simulink model "foc_current_loops"  (R2026b)
settings: Solver=VariableStepAuto  StopTime=6
values from neighbouring files (symbols this model uses):
  D = 5e-5    (= 5e-05)    [setup_foc_current.m]
  J = 0.0239    [setup_foc_current.m]
  Ki_i = 150.0    (= 150)    [setup_foc_current.m]
  Ki_w = 10.0    (= 10)    [setup_foc_current.m]
  Kp_i = 1.5    [setup_foc_current.m]
  Kp_w = 2.0    (= 2)    [setup_foc_current.m]
  L = (Ld + Lq) / 2    (= 0.000225)    [setup_foc_current.m]
  P = 10    [setup_foc_current.m]
  phi_m = 0.05867    [setup_foc_current.m]
  Rs = 25.68e-3    (= 0.02568)    [setup_foc_current.m]
  V_pico = 48    [setup_foc_current.m]
libraries: slpidlib x3, simulink x2
settings Model: Creator=Lemão Som  LastModifiedBy=Lemão Som

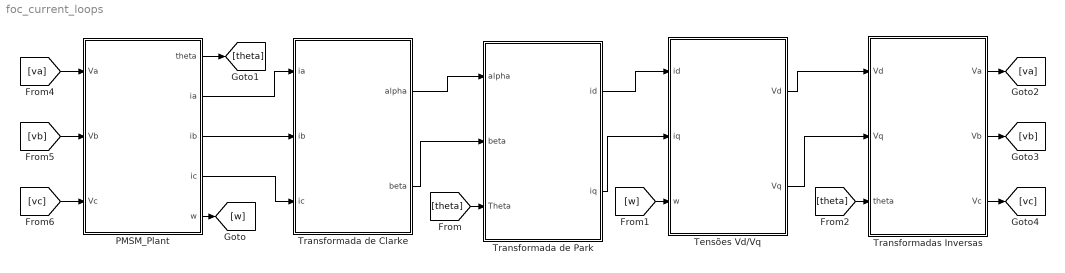
== system foc_current_loops ==
  PMSM_Plant : Subsystem
  Tensões Vd/Vq : Subsystem
  Transformada de Clarke : Subsystem
  Transformada de Park : Subsystem
  Transformadas Inversas : Subsystem
  wires:
  [va] -> PMSM_Plant/1(Va)
  [vb] -> PMSM_Plant/2(Vb)
  [vc] -> PMSM_Plant/3(Vc)
  PMSM_Plant/2(ia) -> Transformada de Clarke/1(ia)
  PMSM_Plant/3(ib) -> Transformada de Clarke/2(ib)
  PMSM_Plant/4(ic) -> Transformada de Clarke/3(ic)
  Transformada de Clarke/1(alpha) -> Transformada de Park/1(alpha)
  PMSM_Plant/5(w) -> [w]
  PMSM_Plant/1(theta) -> [theta]
  [theta] -> Transformada de Park/3(Theta)
  [w] -> Tensões Vd/Vq/3(w)
  Tensões Vd/Vq/1(Vd) -> Transformadas Inversas/1(Vd)
  Tensões Vd/Vq/2(Vq) -> Transformadas Inversas/2(Vq)
  [theta] -> Transformadas Inversas/3(theta)
  Transformadas Inversas/1(Va) -> [va]
  Transformadas Inversas/2(Vb) -> [vb]
  Transformadas Inversas/3(Vc) -> [vc]
  Transformada de Clarke/2(beta) -> Transformada de Park/2(beta)
  Transformada de Park/2(iq) -> Tensões Vd/Vq/2(iq)
  Transformada de Park/1(id) -> Tensões Vd/Vq/1(id)

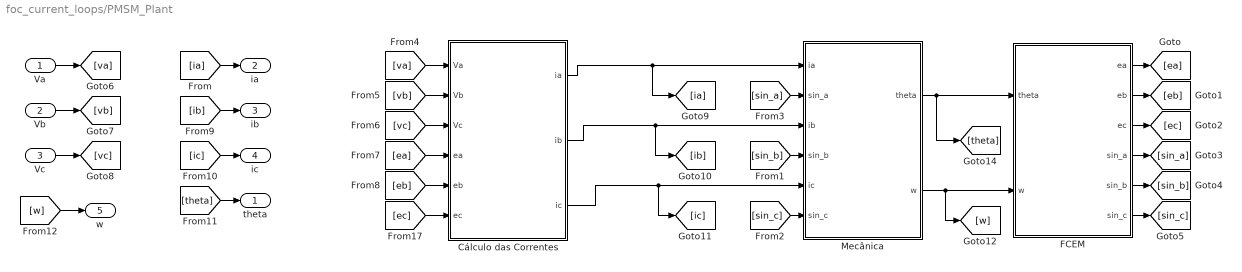
== system foc_current_loops/PMSM_Plant ==
  Va : Inport
  Vb : Inport  Port=2
  Vc : Inport  Port=3
  Cálculo das Correntes : Subsystem
  FCEM : Subsystem
  Mecânica : Subsystem
  theta : Outport
  ia : Outport  Port=2
  ib : Outport  Port=3
  ic : Outport  Port=4
  w : Outport  Port=5
  wires:
  FCEM/2(eb) -> [eb]
  [sin_a] -> Mecânica/2(sin_a)
  [ea] -> Cálculo das Correntes/4(ea)
  [va] -> Cálculo das Correntes/1(Va)
  Cálculo das Correntes/3(ic) -> [ic], Mecânica/5(ic)
  [vb] -> Cálculo das Correntes/2(Vb)
  FCEM/4(sin_a) -> [sin_a]
  FCEM/1(ea) -> [ea]
  Mecânica/1(theta) -> [theta], FCEM/1(theta)
  [vc] -> Cálculo das Correntes/3(Vc)
  FCEM/5(sin_b) -> [sin_b]
  Cálculo das Correntes/2(ib) -> [ib], Mecânica/3(ib)
  Mecânica/2(w) -> [w], FCEM/2(w)
  Cálculo das Correntes/1(ia) -> [ia], Mecânica/1(ia)
  [sin_b] -> Mecânica/4(sin_b)
  [ec] -> Cálculo das Correntes/6(ec)
  [eb] -> Cálculo das Correntes/5(eb)
  FCEM/6(sin_c) -> [sin_c]
  FCEM/3(ec) -> [ec]
  [sin_c] -> Mecânica/6(sin_c)
  Va/1 -> [va]
  Vb/1 -> [vb]
  Vc/1 -> [vc]
  [ia] -> ia/1
  [ib] -> ib/1
  [ic] -> ic/1
  [w] -> w/1
  [theta] -> theta/1

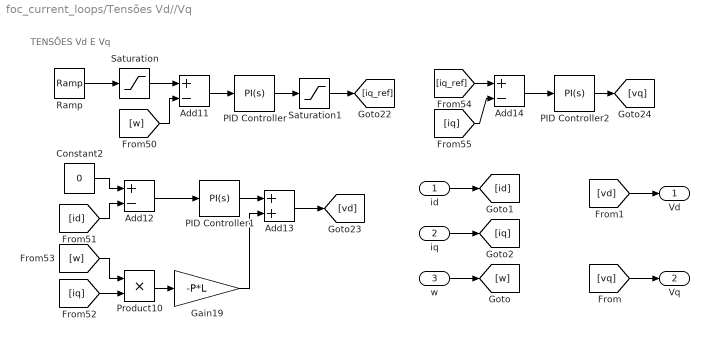
== system foc_current_loops/Tensões Vd//Vq ==
  note: TENSÕES Vd E Vq
  id : Inport
  iq : Inport  Port=2
  w : Inport  Port=3
  Add11 : Sum  Inputs=+-
  Add12 : Sum  Inputs=+-
  Add13 : Sum
  Add14 : Sum  Inputs=+-
  Constant2 : Constant  Value=0
  Gain19 : Gain  Gain=-P*L
  PID Controller : slpidlib/PID Controller  Controller=PI  Form=Parallel  TimeDomain=Continuous-time  UseExternalTs=off  SampleTime=-1  IntegratorMethod=Forward Euler  FilterMethod=Forward Euler  ControllerParametersSource=internal  P=Kp_w  I=Ki_w  UseKiTs=off  D=0  UseExternalDerivativeSource=off  N=100  UseFilter=on  TunerSelectOption=Transfer Function Based (PID Tuner App)  InitialConditionSource=internal  InitialConditionForIntegrator=0  InitialConditionForFilter=0  DifferentiatorICPrevScaledInput=0  ExternalReset=none  TrackingMode=off  Kt=1  LimitOutput=off  SatLimitsSource=internal  UpperSaturationLimit=inf  LowerSaturationLimit=-inf  LinearizeAsGain=on  AntiWindupMode=none  Kb=1  LimitIntegrator=off  UpperIntegratorSaturationLimit=inf  LowerIntegratorSaturationLimit=-inf  POutMin=[]  POutMax=[]  IOutMin=[]  IOutMax=[]  DOutMin=[]  DOutMax=[]  NOutMin=[]  NOutMax=[]  SumOutMin=[]  SumOutMax=[]  SaturationOutMin=[]  SaturationOutMax=[]  PParamMin=[]  PParamMax=[]  IParamMin=[]  IParamMax=[]  DParamMin=[]  DParamMax=[]  NParamMin=[]  NParamMax=[]  KbParamMin=[]  KbParamMax=[]  KtParamMin=[]  KtParamMax=[]  KbOutMin=[]  KbOutMax=[]  KtOutMin=[]  KtOutMax=[]  IntegratorOutMin=[]  IntegratorOutMax=[]  FilterOutMin=[]  FilterOutMax=[]  SumI1OutMin=[]  SumI1OutMax=[]  SumI2OutMin=[]  SumI2OutMax=[]  SumI3OutMin=[]  SumI3OutMax=[]  SumI4OutMin=[]  SumI4OutMax=[]  SumDOutMin=[]  SumDOutMax=[]  DifferentiatorOutMin=[]  DifferentiatorOutMax=[]  FilterDiffOutCoefMin=[]  FilterDiffOutCoefMax=[]  ReciprocalOutMin=[]  ReciprocalOutMax=[]  SumDenOutMin=[]  SumDenOutMax=[]  SumNumOutMin=[]  SumNumOutMax=[]  DivideOutMin=[]  DivideOutMax=[]  UdiffTsProdOutMin=[]  UdiffTsProdOutMax=[]  NTsProdOutMin=[]  NTsProdOutMax=[]  UintegralTsProdOutMin=[]  UintegralTsProdOutMax=[]  UngainTsProdOutMin=[]  UngainTsProdOutMax=[]  ClampingZeroOutDataTypeStr=Inherit: Inherit via back propagation  ClampingZeroOutMin=[]  ClampingZeroOutMax=[]  FilterDenConstantOutDataTypeStr=Inherit: Inherit via back propagation  FilterDenConstantOutMin=[]  FilterDenConstantOutMax=[]  PCopyOutDataTypeStr=Inherit: Inherit via back propagation  PCopyOutMin=[]  PCopyOutMax=[]  NCopyOutDataTypeStr=Inherit: Inherit via back propagation  NCopyOutMin=[]  NCopyOutMax=[]  IntegratorContinuousStateAttributes=''  IntegratorStateMustResolveToSignalObject=off  IntegratorRTWStateStorageClass=Auto  FilterContinuousStateAttributes=''  FilterStateMustResolveToSignalObject=off  FilterRTWStateStorageClass=Auto  ParallelPVariant=InternalParameters  IdealPVariant=Disabled  IVariant=InternalParameters  DVariant=Disabled  IntegratorVariant=Continuous  SatVariant=Disabled  AWVariant=Passthrough  PCopyVariant=Disabled  TRVariant=Disabled  FdbkBlocksVariant=Forward  IdealPFdbkVariant=Disabled  SatFdbkVariant=Disabled  DerivativeFilterVariant=Disabled  NVariant=Disabled  NCopyVariant=Disabled_SignalSpec  FilterICVariant=Disabled  IntegratorICVariant=InternalICs  ExternalResetVariant=Disabled  TRSumVariant=Passthrough  SumFdbkVariant=Disabled  SumVariant=Sum_PI  TsampFilterVariant=InternalTs  TsampNgainVariant=Passthrough  TsampIntegralVariant=Disabled_SignalSpec  ExternalSaturationOutDataTypeStr=Inherit: Same as second input  DerivativeSourceVariant=Disabled  PreIntVariant=InternalPreInt
  PID Controller1 : slpidlib/PID Controller  Controller=PI  Form=Parallel  TimeDomain=Continuous-time  UseExternalTs=off  SampleTime=-1  IntegratorMethod=Forward Euler  FilterMethod=Forward Euler  ControllerParametersSource=internal  P=Kp_i  I=Ki_i  UseKiTs=off  D=0  UseExternalDerivativeSource=off  N=100  UseFilter=on  TunerSelectOption=Transfer Function Based (PID Tuner App)  InitialConditionSource=internal  InitialConditionForIntegrator=0  InitialConditionForFilter=0  DifferentiatorICPrevScaledInput=0  ExternalReset=none  TrackingMode=off  Kt=1  LimitOutput=off  SatLimitsSource=internal  UpperSaturationLimit=inf  LowerSaturationLimit=-inf  LinearizeAsGain=on  AntiWindupMode=none  Kb=1  LimitIntegrator=off  UpperIntegratorSaturationLimit=inf  LowerIntegratorSaturationLimit=-inf  POutMin=[]  POutMax=[]  IOutMin=[]  IOutMax=[]  DOutMin=[]  DOutMax=[]  NOutMin=[]  NOutMax=[]  SumOutMin=[]  SumOutMax=[]  SaturationOutMin=[]  SaturationOutMax=[]  PParamMin=[]  PParamMax=[]  IParamMin=[]  IParamMax=[]  DParamMin=[]  DParamMax=[]  NParamMin=[]  NParamMax=[]  KbParamMin=[]  KbParamMax=[]  KtParamMin=[]  KtParamMax=[]  KbOutMin=[]  KbOutMax=[]  KtOutMin=[]  KtOutMax=[]  IntegratorOutMin=[]  IntegratorOutMax=[]  FilterOutMin=[]  FilterOutMax=[]  SumI1OutMin=[]  SumI1OutMax=[]  SumI2OutMin=[]  SumI2OutMax=[]  SumI3OutMin=[]  SumI3OutMax=[]  SumI4OutMin=[]  SumI4OutMax=[]  SumDOutMin=[]  SumDOutMax=[]  DifferentiatorOutMin=[]  DifferentiatorOutMax=[]  FilterDiffOutCoefMin=[]  FilterDiffOutCoefMax=[]  ReciprocalOutMin=[]  ReciprocalOutMax=[]  SumDenOutMin=[]  SumDenOutMax=[]  SumNumOutMin=[]  SumNumOutMax=[]  DivideOutMin=[]  DivideOutMax=[]  UdiffTsProdOutMin=[]  UdiffTsProdOutMax=[]  NTsProdOutMin=[]  NTsProdOutMax=[]  UintegralTsProdOutMin=[]  UintegralTsProdOutMax=[]  UngainTsProdOutMin=[]  UngainTsProdOutMax=[]  ClampingZeroOutDataTypeStr=Inherit: Inherit via back propagation  ClampingZeroOutMin=[]  ClampingZeroOutMax=[]  FilterDenConstantOutDataTypeStr=Inherit: Inherit via back propagation  FilterDenConstantOutMin=[]  FilterDenConstantOutMax=[]  PCopyOutDataTypeStr=Inherit: Inherit via back propagation  PCopyOutMin=[]  PCopyOutMax=[]  NCopyOutDataTypeStr=Inherit: Inherit via back propagation  NCopyOutMin=[]  NCopyOutMax=[]  IntegratorContinuousStateAttributes=''  IntegratorStateMustResolveToSignalObject=off  IntegratorRTWStateStorageClass=Auto  FilterContinuousStateAttributes=''  FilterStateMustResolveToSignalObject=off  FilterRTWStateStorageClass=Auto  ParallelPVariant=InternalParameters  IdealPVariant=Disabled  IVariant=InternalParameters  DVariant=Disabled  IntegratorVariant=Continuous  SatVariant=Disabled  AWVariant=Passthrough  PCopyVariant=Disabled  TRVariant=Disabled  FdbkBlocksVariant=Forward  IdealPFdbkVariant=Disabled  SatFdbkVariant=Disabled  DerivativeFilterVariant=Disabled  NVariant=Disabled  NCopyVariant=Disabled_SignalSpec  FilterICVariant=Disabled  IntegratorICVariant=InternalICs  ExternalResetVariant=Disabled  TRSumVariant=Passthrough  SumFdbkVariant=Disabled  SumVariant=Sum_PI  TsampFilterVariant=InternalTs  TsampNgainVariant=Passthrough  TsampIntegralVariant=Disabled_SignalSpec  ExternalSaturationOutDataTypeStr=Inherit: Same as second input  DerivativeSourceVariant=Disabled  PreIntVariant=InternalPreInt
  PID Controller2 : slpidlib/PID Controller  Controller=PI  Form=Parallel  TimeDomain=Continuous-time  UseExternalTs=off  SampleTime=-1  IntegratorMethod=Forward Euler  FilterMethod=Forward Euler  ControllerParametersSource=internal  P=Kp_i  I=Ki_i  UseKiTs=off  D=0  UseExternalDerivativeSource=off  N=100  UseFilter=on  TunerSelectOption=Transfer Function Based (PID Tuner App)  InitialConditionSource=internal  InitialConditionForIntegrator=0  InitialConditionForFilter=0  DifferentiatorICPrevScaledInput=0  ExternalReset=none  TrackingMode=off  Kt=1  LimitOutput=off  SatLimitsSource=internal  UpperSaturationLimit=inf  LowerSaturationLimit=-inf  LinearizeAsGain=on  AntiWindupMode=none  Kb=1  LimitIntegrator=off  UpperIntegratorSaturationLimit=inf  LowerIntegratorSaturationLimit=-inf  POutMin=[]  POutMax=[]  IOutMin=[]  IOutMax=[]  DOutMin=[]  DOutMax=[]  NOutMin=[]  NOutMax=[]  SumOutMin=[]  SumOutMax=[]  SaturationOutMin=[]  SaturationOutMax=[]  PParamMin=[]  PParamMax=[]  IParamMin=[]  IParamMax=[]  DParamMin=[]  DParamMax=[]  NParamMin=[]  NParamMax=[]  KbParamMin=[]  KbParamMax=[]  KtParamMin=[]  KtParamMax=[]  KbOutMin=[]  KbOutMax=[]  KtOutMin=[]  KtOutMax=[]  IntegratorOutMin=[]  IntegratorOutMax=[]  FilterOutMin=[]  FilterOutMax=[]  SumI1OutMin=[]  SumI1OutMax=[]  SumI2OutMin=[]  SumI2OutMax=[]  SumI3OutMin=[]  SumI3OutMax=[]  SumI4OutMin=[]  SumI4OutMax=[]  SumDOutMin=[]  SumDOutMax=[]  DifferentiatorOutMin=[]  DifferentiatorOutMax=[]  FilterDiffOutCoefMin=[]  FilterDiffOutCoefMax=[]  ReciprocalOutMin=[]  ReciprocalOutMax=[]  SumDenOutMin=[]  SumDenOutMax=[]  SumNumOutMin=[]  SumNumOutMax=[]  DivideOutMin=[]  DivideOutMax=[]  UdiffTsProdOutMin=[]  UdiffTsProdOutMax=[]  NTsProdOutMin=[]  NTsProdOutMax=[]  UintegralTsProdOutMin=[]  UintegralTsProdOutMax=[]  UngainTsProdOutMin=[]  UngainTsProdOutMax=[]  ClampingZeroOutDataTypeStr=Inherit: Inherit via back propagation  ClampingZeroOutMin=[]  ClampingZeroOutMax=[]  FilterDenConstantOutDataTypeStr=Inherit: Inherit via back propagation  FilterDenConstantOutMin=[]  FilterDenConstantOutMax=[]  PCopyOutDataTypeStr=Inherit: Inherit via back propagation  PCopyOutMin=[]  PCopyOutMax=[]  NCopyOutDataTypeStr=Inherit: Inherit via back propagation  NCopyOutMin=[]  NCopyOutMax=[]  IntegratorContinuousStateAttributes=''  IntegratorStateMustResolveToSignalObject=off  IntegratorRTWStateStorageClass=Auto  FilterContinuousStateAttributes=''  FilterStateMustResolveToSignalObject=off  FilterRTWStateStorageClass=Auto  ParallelPVariant=InternalParameters  IdealPVariant=Disabled  IVariant=InternalParameters  DVariant=Disabled  IntegratorVariant=Continuous  SatVariant=Disabled  AWVariant=Passthrough  PCopyVariant=Disabled  TRVariant=Disabled  FdbkBlocksVariant=Forward  IdealPFdbkVariant=Disabled  SatFdbkVariant=Disabled  DerivativeFilterVariant=Disabled  NVariant=Disabled  NCopyVariant=Disabled_SignalSpec  FilterICVariant=Disabled  IntegratorICVariant=InternalICs  ExternalResetVariant=Disabled  TRSumVariant=Passthrough  SumFdbkVariant=Disabled  SumVariant=Sum_PI  TsampFilterVariant=InternalTs  TsampNgainVariant=Passthrough  TsampIntegralVariant=Disabled_SignalSpec  ExternalSaturationOutDataTypeStr=Inherit: Same as second input  DerivativeSourceVariant=Disabled  PreIntVariant=InternalPreInt
  Product10 : Product
  Ramp : simulink/Sources/Ramp  slope=600  start=0  InitialOutput=0
  Saturation : Saturate  UpperLimit=300  LowerLimit=0
  Saturation1 : Saturate  UpperLimit=250  LowerLimit=-250
  Vd : Outport
  Vq : Outport  Port=2
  wires:
  Add11/1 -> PID Controller/1
  PID Controller2/1 -> [vq]
  Saturation/1 -> Add11/1
  [id] -> Add12/2
  [w] -> Product10/1
  Product10/1 -> Gain19/1
  PID Controller/1 -> Saturation1/1
  [iq] -> Add14/2
  [iq] -> Product10/2
  Add13/1 -> [vd]
  [iq_ref] -> Add14/1
  Add14/1 -> PID Controller2/1
  [w] -> Add11/2
  Gain19/1 -> Add13/2
  PID Controller1/1 -> Add13/1
  Ramp/1 -> Saturation/1
  Add12/1 -> PID Controller1/1
  Constant2/1 -> Add12/1
  Saturation1/1 -> [iq_ref]
  w/1 -> [w]
  id/1 -> [id]
  iq/1 -> [iq]
  [vq] -> Vq/1
  [vd] -> Vd/1

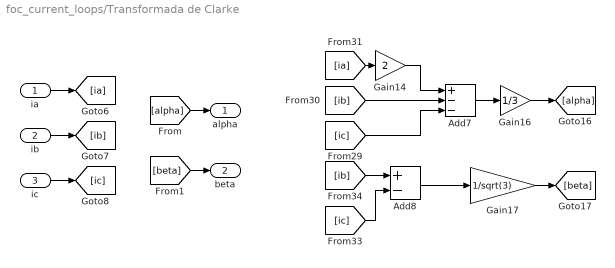
== system foc_current_loops/Transformada de Clarke ==
  ia : Inport
  ib : Inport  Port=2
  ic : Inport  Port=3
  Add7 : Sum  Inputs=+--
  Add8 : Sum  Inputs=+-
  Gain14 : Gain  Gain=2
  Gain16 : Gain  Gain=1/3
  Gain17 : Gain  Gain=1/sqrt(3)
  alpha : Outport
  beta : Outport  Port=2
  wires:
  ic/1 -> [ic]
  ib/1 -> [ib]
  ia/1 -> [ia]
  Gain14/1 -> Add7/1
  [ib] -> Add8/1
  Gain16/1 -> [alpha]
  [ic] -> Add7/3
  Gain17/1 -> [beta]
  [ic] -> Add8/2
  [ia] -> Gain14/1
  Add8/1 -> Gain17/1
  Add7/1 -> Gain16/1
  [ib] -> Add7/2
  [alpha] -> alpha/1
  [beta] -> beta/1

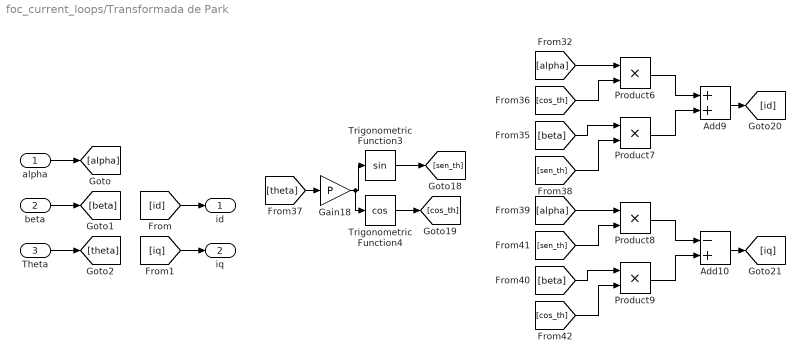
== system foc_current_loops/Transformada de Park ==
  alpha : Inport
  beta : Inport  Port=2
  Theta : Inport  Port=3
  Add10 : Sum  Inputs=-+
  Add9 : Sum
  Gain18 : Gain  Gain=P
  Product{6..9} (4 alike) : Product
  Trigonometric Function3 : Trigonometry
  Trigonometric Function4 : Trigonometry  Operator=cos
  id : Outport
  iq : Outport  Port=2
  wires:
  [iq] -> iq/1
  Theta/1 -> [theta]
  Add10/1 -> [iq]
  Add9/1 -> [id]
  Product7/1 -> Add9/2
  Product6/1 -> Add9/1
  [sen_th] -> Product8/2
  [sen_th] -> Product7/2
  [alpha] -> Product6/1
  [beta] -> Product9/1
  [theta] -> Gain18/1
  Product9/1 -> Add10/2
  Gain18/1 -> Trigonometric Function4/1, Trigonometric Function3/1
  [cos_th] -> Product9/2
  [beta] -> Product7/1
  Trigonometric Function4/1 -> [cos_th]
  alpha/1 -> [alpha]
  [alpha] -> Product8/1
  beta/1 -> [beta]
  [id] -> id/1
  Product8/1 -> Add10/1
  [cos_th] -> Product6/2
  Trigonometric Function3/1 -> [sen_th]

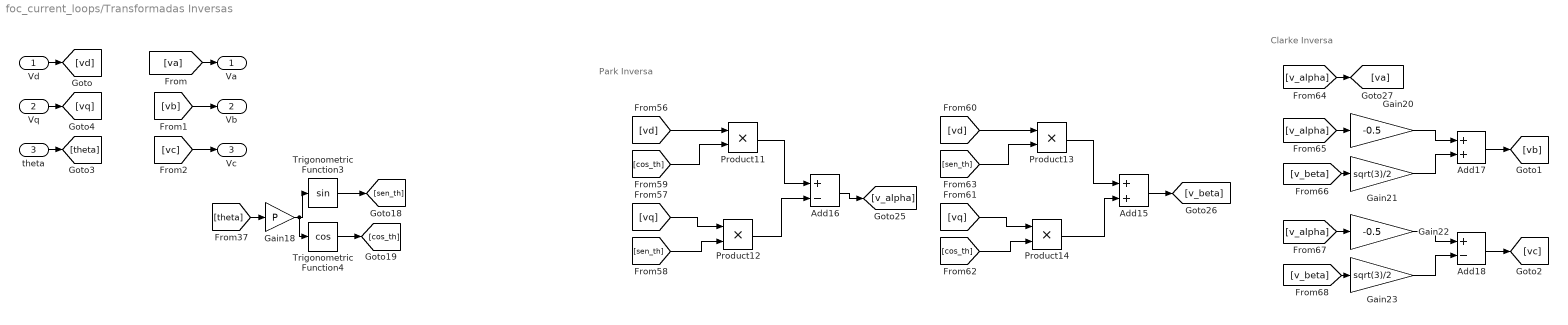
== system foc_current_loops/Transformadas Inversas ==
  note: Clarke Inversa
  note: Park Inversa
  Vd : Inport
  Vq : Inport  Port=2
  theta : Inport  Port=3
  Add15 : Sum
  Add16 : Sum  Inputs=+-
  Add17 : Sum
  Add18 : Sum  Inputs=+-
  Gain18 : Gain  Gain=P
  Gain20 : Gain  Gain=-0.5
  Gain21 : Gain  Gain=sqrt(3)/2
  Gain22 : Gain  Gain=-0.5
  Gain23 : Gain  Gain=sqrt(3)/2
  Product{11..14} (4 alike) : Product
  Trigonometric Function3 : Trigonometry
  Trigonometric Function4 : Trigonometry  Operator=cos
  Va : Outport
  Vb : Outport  Port=2
  Vc : Outport  Port=3
  wires:
  Add15/1 -> [v_beta]
  [cos_th] -> Product11/2
  Gain21/1 -> Add17/2
  [v_alpha] -> Gain22/1
  Add16/1 -> [v_alpha]
  [sen_th] -> Product13/2
  Product11/1 -> Add16/1
  Add18/1 -> [vc]
  [vd] -> Product11/1
  [vd] -> Product13/1
  [v_alpha] -> Gain20/1
  Gain23/1 -> Add18/2
  Gain20/1 -> Add17/1
  Gain22/1 -> Add18/1
  Product12/1 -> Add16/2
  Product14/1 -> Add15/2
  [v_beta] -> Gain21/1
  [vq] -> Product12/1
  [vq] -> Product14/1
  [sen_th] -> Product12/2
  [v_beta] -> Gain23/1
  [v_alpha] -> [va]
  Product13/1 -> Add15/1
  [cos_th] -> Product14/2
  Add17/1 -> [vb]
  Trigonometric Function3/1 -> [sen_th]
  Gain18/1 -> Trigonometric Function4/1, Trigonometric Function3/1
  [theta] -> Gain18/1
  Trigonometric Function4/1 -> [cos_th]
  Vd/1 -> [vd]
  theta/1 -> [theta]
  Vq/1 -> [vq]
  [va] -> Va/1
  [vb] -> Vb/1
  [vc] -> Vc/1

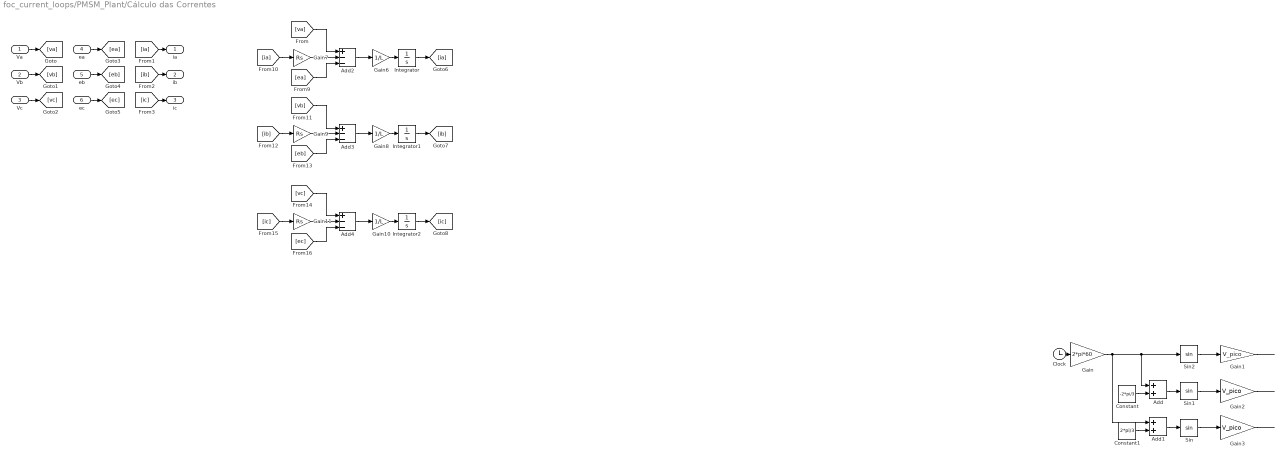
== system foc_current_loops/PMSM_Plant/Cálculo das Correntes ==
  Va : Inport
  Vb : Inport  Port=2
  Vc : Inport  Port=3
  ea : Inport  Port=4
  eb : Inport  Port=5
  ec : Inport  Port=6
  Add : Sum
  Add1 : Sum
  Add2 : Sum  Inputs=+--
  Add3 : Sum  Inputs=+--
  Add4 : Sum  Inputs=+--
  Clock : Clock
  Constant : Constant  Value=-2*pi/3
  Constant1 : Constant  Value=2*pi/3
  Gain : Gain  Gain=2*pi*60
  Gain1 : Gain  Gain=V_pico
  Gain10 : Gain  Gain=1/L
  Gain11 : Gain  Gain=Rs
  Gain2 : Gain  Gain=V_pico
  Gain3 : Gain  Gain=V_pico
  Gain6 : Gain  Gain=1/L
  Gain7 : Gain  Gain=Rs
  Gain8 : Gain  Gain=1/L
  Gain9 : Gain  Gain=Rs
  Integrator : Integrator
  Integrator1 : Integrator
  Integrator2 : Integrator
  Sin : Trigonometry
  Sin1 : Trigonometry
  Sin2 : Trigonometry
  ia : Outport
  ib : Outport  Port=2
  ic : Outport  Port=3
  wires:
  Sin/1 -> Gain3/1
  Clock/1 -> Gain/1
  Gain1/1 -> ?
  Sin1/1 -> Gain2/1
  Gain2/1 -> ?
  Add1/1 -> Sin/1
  Sin2/1 -> Gain1/1
  Gain/1 -> Add/1, Sin2/1, Add1/1
  Gain3/1 -> ?
  Add/1 -> Sin1/1
  Constant/1 -> Add/2
  Constant1/1 -> Add1/2
  Integrator2/1 -> [ic]
  [ea] -> Add2/3
  [ec] -> Add4/3
  Add3/1 -> Gain8/1
  [eb] -> Add3/3
  Integrator1/1 -> [ib]
  Gain7/1 -> Add2/2
  Gain8/1 -> Integrator1/1
  Add4/1 -> Gain10/1
  Add2/1 -> Gain6/1
  Gain10/1 -> Integrator2/1
  [va] -> Add2/1
  [ic] -> Gain11/1
  Gain9/1 -> Add3/2
  [ia] -> Gain7/1
  Integrator/1 -> [ia]
  Gain11/1 -> Add4/2
  [vc] -> Add4/1
  [vb] -> Add3/1
  Gain6/1 -> Integrator/1
  [ib] -> Gain9/1
  Va/1 -> [va]
  Vb/1 -> [vb]
  Vc/1 -> [vc]
  ea/1 -> [ea]
  eb/1 -> [eb]
  ec/1 -> [ec]
  [ib] -> ib/1
  [ic] -> ic/1
  [ia] -> ia/1

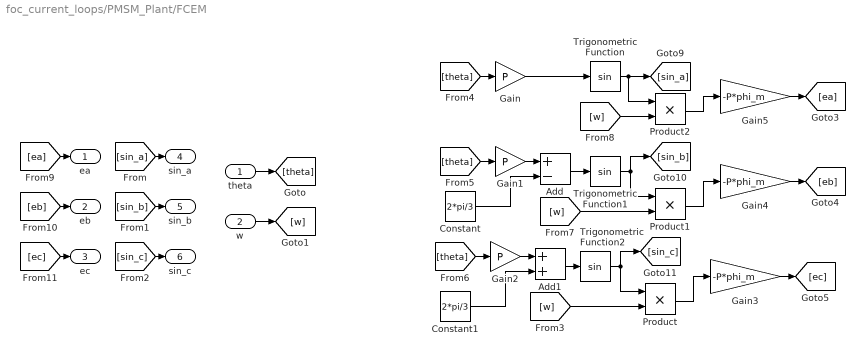
== system foc_current_loops/PMSM_Plant/FCEM ==
  theta : Inport
  w : Inport  Port=2
  Add : Sum  Inputs=+-
  Add1 : Sum
  Constant : Constant  Value=2*pi/3
  Constant1 : Constant  Value=2*pi/3
  Gain : Gain  Gain=P
  Gain1 : Gain  Gain=P
  Gain2 : Gain  Gain=P
  Gain3 : Gain  Gain=-P*phi_m
  Gain4 : Gain  Gain=-P*phi_m
  Gain5 : Gain  Gain=-P*phi_m
  Product : Product
  Product1 : Product
  Product2 : Product
  Trigonometric Function : Trigonometry
  Trigonometric Function1 : Trigonometry
  Trigonometric Function2 : Trigonometry
  ea : Outport
  eb : Outport  Port=2
  ec : Outport  Port=3
  sin_a : Outport  Port=4
  sin_b : Outport  Port=5
  sin_c : Outport  Port=6
  wires:
  Product1/1 -> Gain4/1
  Gain5/1 -> [ea]
  Gain1/1 -> Add/1
  [theta] -> Gain/1
  Constant/1 -> Add/2
  Constant1/1 -> Add1/2
  Gain2/1 -> Add1/1
  Trigonometric Function/1 -> Product2/1, [sin_a]
  Trigonometric Function1/1 -> [sin_b], Product1/1
  Gain/1 -> Trigonometric Function/1
  Product/1 -> Gain3/1
  [w] -> Product2/2
  [w] -> Product1/2
  [theta] -> Gain1/1
  Add1/1 -> Trigonometric Function2/1
  Gain4/1 -> [eb]
  [theta] -> Gain2/1
  [w] -> Product/2
  Gain3/1 -> [ec]
  Product2/1 -> Gain5/1
  Add/1 -> Trigonometric Function1/1
  Trigonometric Function2/1 -> [sin_c], Product/1
  theta/1 -> [theta]
  w/1 -> [w]
  [ea] -> ea/1
  [eb] -> eb/1
  [ec] -> ec/1
  [sin_c] -> sin_c/1
  [sin_b] -> sin_b/1
  [sin_a] -> sin_a/1

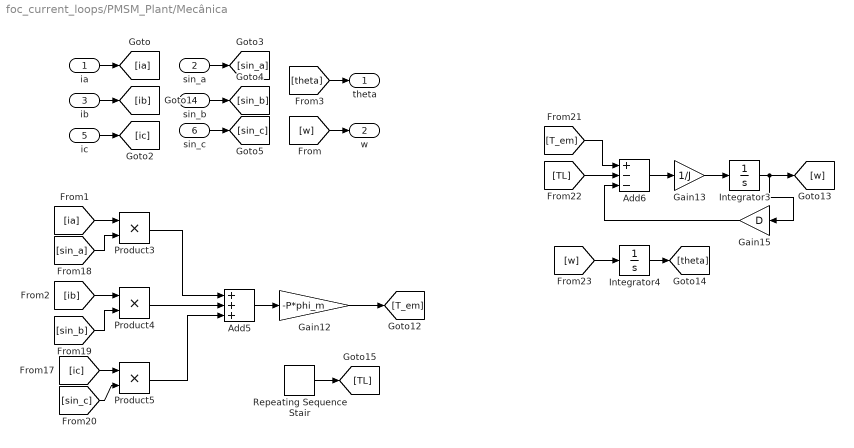
== system foc_current_loops/PMSM_Plant/Mecânica ==
  ia : Inport
  sin_a : Inport  Port=2
  ib : Inport  Port=3
  sin_b : Inport  Port=4
  ic : Inport  Port=5
  sin_c : Inport  Port=6
  Add5 : Sum  Inputs=+++
  Add6 : Sum  Inputs=+--
  Gain12 : Gain  Gain=-P*phi_m
  Gain13 : Gain  Gain=1/J
  Gain15 : Gain  Gain=D
  Integrator3 : Integrator
  Integrator4 : Integrator
  Product3 : Product
  Product4 : Product
  Product5 : Product
  Repeating Sequence Stair : simulink/Sources/Repeating Sequence Stair  OutValues=[0, 0, 30, 60, 20, 0]  tsamp=1  OutMin=[]  OutMax=[]  OutDataTypeStr=double  OutputDataTypeScalingMode=double  OutDataType=fixdt(0,8)  ConRadixGroup=Best Precision: Vector-wise  OutScaling=2^-12
  theta : Outport
  w : Outport  Port=2
  wires:
  ic/1 -> [ic]
  ib/1 -> [ib]
  ia/1 -> [ia]
  [T_em] -> Add6/1
  [w] -> Integrator4/1
  [ia] -> Product3/1
  [ib] -> Product4/1
  [ic] -> Product5/1
  Product5/1 -> Add5/3
  [sin_b] -> Product4/2
  Integrator3/1 -> Gain15/1, [w]
  Gain15/1 -> Add6/3
  [sin_c] -> Product5/2
  [sin_a] -> Product3/2
  Add6/1 -> Gain13/1
  Add5/1 -> Gain12/1
  Integrator4/1 -> [theta]
  Gain13/1 -> Integrator3/1
  Repeating Sequence Stair/1 -> [TL]
  Product3/1 -> Add5/1
  [TL] -> Add6/2
  Gain12/1 -> [T_em]
  Product4/1 -> Add5/2
  sin_a/1 -> [sin_a]
  sin_b/1 -> [sin_b]
  sin_c/1 -> [sin_c]
  [theta] -> theta/1
  [w] -> w/1
